simulink model "Example_1DAC_2ADC"  (R2023b)
settings: Solver=VariableStepAuto  StartTime=0.0  StopTime=2.0e-3  RelTol=1e-3
settings Model: Creator=rlschie  LastModifiedBy=rlschie
settings DebuggingCC: UnconnectedInputMsg=warning  UnconnectedOutputMsg=warning  UnconnectedLineMsg=warning
settings ModelReferenceCC: EnableRefExpFcnMdlSchedulingChecks=on
settings RTWCC: DLArmComputeVersion=19.05

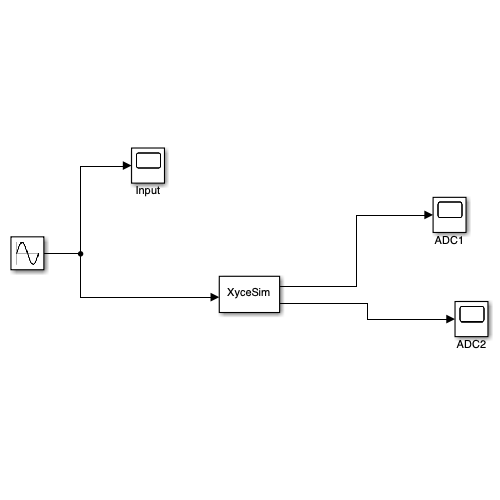
[thumbnail: Simulink's stored preview of the top-level diagram]
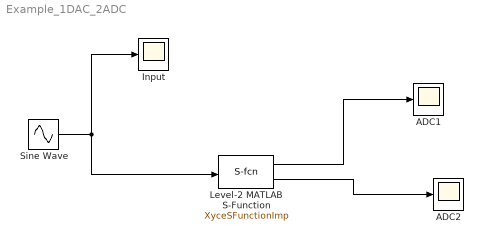
== system Example_1DAC_2ADC ==
  ADC1 : Scope
  ADC2 : Scope
  Input : Scope
  Level-2 MATLAB S-Function : M-S-Function  FunctionName=XyceSFunctionImp  Parameters=XyceInputFileName,WorkingDirectory,NumberOfInputs,NumberOfOutputs,InputNames,OutputNames  mask{XyceInputFileName=1Dac2ADCSystem.cir, WorkingDirectory=/Users/rlschie/src/XyceDevelopment/Xyce/utils/SimulinkInterface/SimulinkExamples/, XyceInputPortNames=, XyceOutputPortNames=, XyceNumberOfInputPorts=0, XyceNumberOfOutputPorts=0, NumberOfInputs=1, NumberOfOutputs=2, InputNames={ '1', 'YDAC!DAC_DRIVER1' }, OutputNames={ '2', 'YADC!ADC2'; '1', 'YADC!ADC1' }}
      mask prompts: XyceInputFileName "Xyce Input Filename"; WorkingDirectory "Working Directory"; XyceInputPortNames "Xyce Input Port Names"; XyceOutputPortNames "Xyce Output Port Names"; XyceNumberOfInputPorts "Xyce Number Of Inputs"; XyceNumberOfOutputPorts "Xyce Number Of Outputs"; NumberOfInputs "Number of Inputs"; NumberOfOutputs "Number of Outputs"; InputNames "Input Names"; OutputNames "Output Names"
      mask DialogControl SelectXyceInputFileButton Prompt: Select Xyce Input File
      mask DialogControl ScanXyceInputFileButton Prompt: Scan Xyce Input File
      mask DialogControl ResetForm Prompt: Reset
      mask DialogControl AddInputLineButton Prompt: Add Line
      mask DialogControl RemoveInputLineButton Prompt: Remove Line
      mask DialogControl AddOutputLineButton Prompt: Add Line
      mask DialogControl RemoveOutputLineButton Prompt: Remove Line
      mask Display: disp('XyceSim');
  Sine Wave : Sin  Frequency=3000  SampleTime=0
  wires:
  Sine Wave/1 -> Level-2 MATLAB S-Function/1, Input/1
  Level-2 MATLAB S-Function/1 -> ADC1/1
  Level-2 MATLAB S-Function/2 -> ADC2/1
